simulink model "compare_process_models.slx"  (R2024b)
settings: Solver=VariableStepAuto  StartTime=0.0  StopTime=100  RelTol=1e-3
settings Model: Creator=bashi  LastModifiedBy=bashi

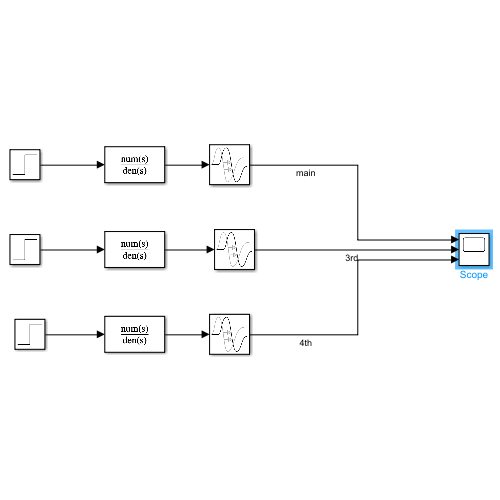
[thumbnail: Simulink's stored preview of the top-level diagram]
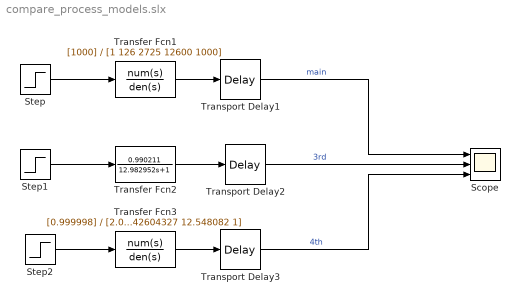
== system compare_process_models.slx ==
  Scope : Scope  NumInputPorts=3
  Step : Step  SampleTime=0
  Step1 : Step  SampleTime=0
  Step2 : Step  SampleTime=0
  Transfer Fcn1 : TransferFcn  Numerator=[1000]  Denominator=[1 126 2725 12600 1000]
  Transfer Fcn2 : TransferFcn  Numerator=[0.990211]  Denominator=[12.982952 1]
  Transfer Fcn3 : TransferFcn  Numerator=[0.999998]  Denominator=[2.0742604327 12.548082 1]
  Transport Delay1 : TransportDelay  DelayTime=2.5
  Transport Delay2 : TransportDelay  DelayTime=2.698647
  Transport Delay3 : TransportDelay  DelayTime=2.551851
  wires:
  Step/1 -> Transfer Fcn1/1
  Transfer Fcn1/1 -> Transport Delay1/1
  Transport Delay1/1 -> Scope/1  "main"
  Transfer Fcn2/1 -> Transport Delay2/1
  Step1/1 -> Transfer Fcn2/1
  Transfer Fcn3/1 -> Transport Delay3/1
  Step2/1 -> Transfer Fcn3/1
  Transport Delay2/1 -> Scope/2  "3rd"
  Transport Delay3/1 -> Scope/3  "4th"
